simulink model "System_Model_Draft"  (R2025b)
settings: Solver=VariableStepAuto  StartTime=0.0  StopTime=10.0  RelTol=1e-3
libraries: matrix_library x2
settings Model: Creator=User  LastModifiedBy=User

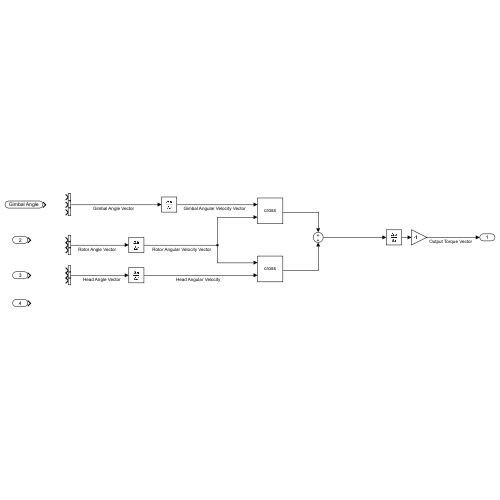
[thumbnail: Simulink's stored preview of the top-level diagram]
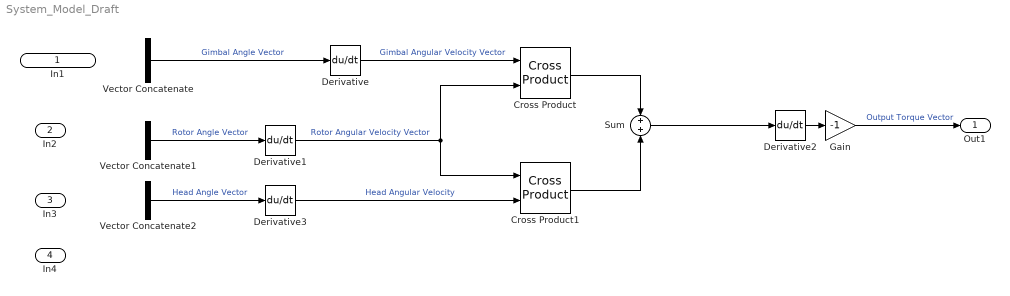
== system System_Model_Draft ==
  In1 : Inport
  In2 : Inport  Port=2
  In3 : Inport  Port=3
  In4 : Inport  Port=4
  Cross Product : matrix_library/Cross Product
  Cross Product1 : matrix_library/Cross Product
  Derivative{,1..3} (4 alike) : Derivative
  Gain : Gain  Gain=-1
  Sum : Sum  Inputs=+|+
  Vector Concatenate : Concatenate  NumInputs=3
  Vector Concatenate1 : Concatenate  NumInputs=3
  Vector Concatenate2 : Concatenate  NumInputs=3
  Out1 : Outport
  wires:
  Vector Concatenate/1 -> Derivative/1  "Gimbal Angle Vector"
  Derivative/1 -> Cross Product/1  "Gimbal Angular Velocity Vector"
  Vector Concatenate1/1 -> Derivative1/1  "Rotor Angle Vector"
  Derivative1/1 -> Cross Product/2, Cross Product1/1  "Rotor Angular Velocity Vector"
  Derivative2/1 -> Gain/1
  Gain/1 -> Out1/1  "Output Torque Vector"
  Vector Concatenate2/1 -> Derivative3/1  "Head Angle Vector"
  Derivative3/1 -> Cross Product1/2  "Head Angular Velocity"
  Cross Product/1 -> Sum/1
  Cross Product1/1 -> Sum/2
  Sum/1 -> Derivative2/1
